simulink model "example_of_using"  (R2023b)
settings: Solver=VariableStepAuto  StartTime=0.0  StopTime=inf  RelTol=1e-3
settings Model: Creator=levadny  LastModifiedBy=levadny

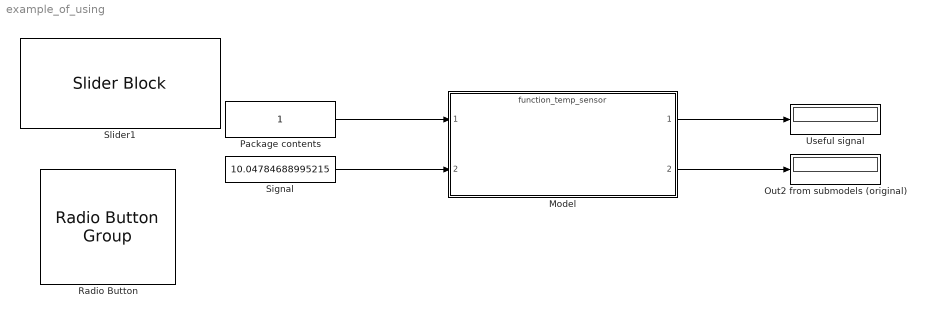
== system example_of_using ==
  Model : ModelReference  ModelNameDialog=function_temp_sensor.slx  SimulationMode=Normal  ModelReferenceVersion=1.30
  Out2 from submodels (original) : Display
  Package contents : Constant  OutDataTypeStr=int8
  Radio Button : RadioButtonGroup  SelectedLabel=Log  ButtonGroupName=Group
      settings: Values={{'Not', 'Log', 'Exp', 'Square'}, [0 1 2 3]}
  Signal : Constant  Value=10.04784688995215  OutDataTypeStr=double
  Slider1 : SliderBlock  TickInterval=10
  Useful signal : Display
  wires:
  Model/1 -> Useful signal/1
  Model/2 -> Out2 from submodels (original)/1
  Signal/1 -> Model/2
  Package contents/1 -> Model/1
